simulink model "UAV_SIMULATOR_CA_2021a"  (R2024a)
settings: Solver=FixedStepAuto  StartTime=0.0  StopTime=tf_echelons  FixedStep=0.002  RelTol=1e-4
values from neighbouring files (symbols this model uses):
  Beta_OPT = [Beta, Z_max: 0.1*pi/180: betaf]    [UAV_SIMULATOR_MAIN_0.m]
  betaf = 20*pi/180 +betai    (= 0.660268528005)    [UAV_SIMULATOR_MAIN_0.m]
  betai = 17.8306*pi/180    (= 0.311202677606)    [UAV_SIMULATOR_MAIN_0.m]
  Bp_offset = 0.06    [UAV_SIMULATOR_MAIN_0.m]
  CDy = data(1)    [Aero_initial.m]    (also in FunLagragian.m; UAV_SIMULATOR_MAIN_0.m = 1; costFunction.m; nonLinearConstraints.m)
  CLOSED_LOOP_ESCs = 1    [UAV_SIMULATOR_MAIN_0.m]
  cQ = 2.1113*1e-08    (= 2.1113e-08)    [UAV_SIMULATOR_MAIN_0.m]
  cQ_Magnus = 0.5*S/2*RM^3*Cf    (= 4.804078125e-10)    [UAV_SIMULATOR_MAIN_0.m]
  cT = 2.4815e-6    (= 2.4815e-06)    [UAV_SIMULATOR_MAIN_0.m]
  cT_1_6 = 2.1030e-06    (= 2.103e-06)    [UAV_SIMULATOR_MAIN_0.m]
  D_PQR_PX4 = diag([D_ROLL D_PITCH D_YAW])    [UAV_SIMULATOR_MAIN_0.m]
  ethaf = 25*pi/180    (= 0.436332312999)    [UAV_SIMULATOR_MAIN_0.m]
  ethai = 0 *pi/180    (= 0)    [UAV_SIMULATOR_MAIN_0.m]
  F_fric = 0.5    [UAV_SIMULATOR_MAIN_0.m]
  Fa_L_int = Rmat*(FaG_int+FaG_int_d)    [UAV_SIMULATOR_MAIN_0.m]
  g = data(7)    [FunLagragian.m]    (also in UAV_SIMULATOR_MAIN_0.m = 9.81; costFunction.m; nonLinearConstraints.m; runOptimizationHelper.m = comp(7))
  I_PQR_PX4 = diag([I_ROLL I_PITCH I_YAW])    [UAV_SIMULATOR_MAIN_0.m]
  initial_attitude_condition = 1*[0 0 pi]    [UAV_SIMULATOR_MAIN_0.m]
  initial_pos_conditions = [ri*cos(betai) 0 ri*sin(betai) + Bp_offset]    [UAV_SIMULATOR_MAIN_0.m]
  Jr = 1.2991*1e-05    (= 1.2991e-05)    [UAV_SIMULATOR_MAIN_0.m]
  Jr_Magnus = JM1(2,2)    [UAV_SIMULATOR_MAIN_0.m]
  K_DI_int = [diag([k_r(1), k_etha(1), k_beta(1)]), diag([k_r(2), k_etha(2), k_beta(2)]), diag([k_r(3), k_etha(3), k_beta(3)])]    [UAV_SIMULATOR_MAIN_0.m]
  K_PQR_PX4 = 1*diag([0.8 1.35 1])    [UAV_SIMULATOR_MAIN_0.m]
  km = 1/Kv_motor_rad    (= 0.00545674090601)    [UAV_SIMULATOR_MAIN_0.m]
  L = lqr(A,B,Q_beta,R_beta)    [UAV_SIMULATOR_MAIN_0.m]
  L_mot = 1.0000e-04    (= 0.0001)    [UAV_SIMULATOR_MAIN_0.m]
  LM = 0.28*2    (= 0.56)    [UAV_SIMULATOR_MAIN_0.m]
  m = data(6)    [FunLagragian.m]    (also in UAV_SIMULATOR_MAIN_0.m = 1.746; costFunction.m; nonLinearConstraints.m; runOptimizationHelper.m = comp(6))
  m_M1 = 0.049    [UAV_SIMULATOR_MAIN_0.m]
  m_M2 = 0.049    [UAV_SIMULATOR_MAIN_0.m]
  m_w = 0.0481    [UAV_SIMULATOR_MAIN_0.m]    (also in nonLinearConstraints.m = data(9); runOptimizationHelper.m = comp(9))
  max_angle = max_angle_deg*pi/180    (= 0.610865238198)    [UAV_SIMULATOR_MAIN_0.m]
  nb_battery_cells = 4    [UAV_SIMULATOR_MAIN_0.m]
  P_ATTITUDE_PX4 = diag([10 10 2.8])    [UAV_SIMULATOR_MAIN_0.m]
  P_PQR_PX4 = diag([P_ROLL P_PITCH P_YAW])    [UAV_SIMULATOR_MAIN_0.m]
  PX4_attitude_loop_frequency = 250    [UAV_SIMULATOR_MAIN_0.m]
  PX4_rate_loop_frequency = 500    [UAV_SIMULATOR_MAIN_0.m]
  R = data(4)    [Aero_initial.m]    (also in UAV_SIMULATOR_MAIN_0.m = 0.07)
  R_bat = 0.024    [UAV_SIMULATOR_MAIN_0.m]
  rf = 1.5    [UAV_SIMULATOR_MAIN_0.m]
  rho_air = data(8)    [FunLagragian.m]    (also in UAV_SIMULATOR_MAIN_0.m = 1.293; costFunction.m; nonLinearConstraints.m; runOptimizationHelper.m = comp(8))
  ri = 0.490142    [UAV_SIMULATOR_MAIN_0.m]
  RM = data(4)    [FunLagragian.m]    (also in UAV_SIMULATOR_MAIN_0.m = 0.0275; costFunction.m; nonLinearConstraints.m; runOptimizationHelper.m = comp(4))
  S = data(3)    [Aero_initial.m]    (also in FunLagragian.m; UAV_SIMULATOR_MAIN_0.m = 0.0308; costFunction.m; nonLinearConstraints.m)
  s_M1D = [0, LM/4, 0]'    [UAV_SIMULATOR_MAIN_0.m]
  s_M2D = [0, -LM/4, 0]'    [UAV_SIMULATOR_MAIN_0.m]
  Slat = data(2)    [Aero_initial.m]    (also in FunLagragian.m; UAV_SIMULATOR_MAIN_0.m = 0.00237582944428; costFunction.m; nonLinearConstraints.m)
  state_int = [0 0 0 initial_attitude_condition 0 0 0 initial_attitude_quaternion_condition]    [UAV_SIMULATOR_MAIN_0.m]
  T0 = 1.5    [UAV_SIMULATOR_MAIN_0.m]
  t0 = 0    [UAV_SIMULATOR_MAIN_0.m]
  t1 = t0 + 15    (= 15)    [UAV_SIMULATOR_MAIN_0.m]
  t1T = t1/10    (= 1.5)    [UAV_SIMULATOR_MAIN_0.m]
  t2 = t1 + 15    (= 30)    [UAV_SIMULATOR_MAIN_0.m]    (also in plot_test.m = Simulation_Data.time)
  t2T = t2 + 9*t1/10    (= 43.5)    [UAV_SIMULATOR_MAIN_0.m]
  t3 = t2 + 15    (= 45)    [UAV_SIMULATOR_MAIN_0.m]
  tau_ur_model = 0.001    [UAV_SIMULATOR_MAIN_0.m]
  Tf = 1.5    [UAV_SIMULATOR_MAIN_0.m]
  Ti = 0    [UAV_SIMULATOR_MAIN_0.m]
  Ts = 0.02    [UAV_SIMULATOR_MAIN_0.m]
  U_sat = 3.7*nb_battery_cells    (= 14.8)    [UAV_SIMULATOR_MAIN_0.m]
  ViconTracker_noise_mean = 0.00001    (= 1e-05)    [UAV_SIMULATOR_MAIN_0.m]
  ViconTracker_noise_variance = 0.000001    (= 1e-06)    [UAV_SIMULATOR_MAIN_0.m]
  vitesse_vent = [0, 0, 0]'    [UAV_SIMULATOR_MAIN_0.m]
  vmag = 0    [UAV_SIMULATOR_MAIN_0.m]
  vx_wind = [vwind(1,1:t_winddirc_change/dt-1) vx_inter vwind(1,(t_winddirc_change+1)/dt +1:final_time/dt+1)*cos(10*pi/180)]    [UAV_SIMULATOR_MAIN_0.m]
  vy_wind = [zeros(1,t_winddirc_change/dt-1) vy_inter vwind(1,(t_winddirc_change+1)/dt +1:final_time/dt+1)*sin(10*pi/180)]    [UAV_SIMULATOR_MAIN_0.m]
  wind_turb = 1    [UAV_SIMULATOR_MAIN_0.m]
  wn_beta = 2    [UAV_SIMULATOR_MAIN_0.m]
  wn_etha = 2    [UAV_SIMULATOR_MAIN_0.m]
  wn_r = 2    [UAV_SIMULATOR_MAIN_0.m]
  X0 = 4    [UAV_SIMULATOR_MAIN_0.m]    (also in runOptimizationHelper.m = data(19))
  X1 = min(X1,8)    [Aero_initial.m]    (also in UAV_SIMULATOR_MAIN_0.m = [X1, X1(end)])
undefined symbols (not defined in the file or in its folder): DiscIntNeverNeededParam, PWM_data_map
libraries: simulink x23, slpidlib x5, eeGeneralControl x3, simulink_extras x1
(part 1 of 3)
settings Model: Creator=admin  LastModifiedBy=Abdelateef
settings DataIOCC: ReturnWorkspaceOutputs=off
settings DebuggingCC: UnconnectedInputMsg=warning  UnconnectedOutputMsg=warning  UnconnectedLineMsg=warning  ArithmeticOperatorsInVariantConditions=warning
settings ModelReferenceCC: EnableRefExpFcnMdlSchedulingChecks=on
settings SFSimCC: SimCustomHeaderCode=calculateOptimizedMagnusAndResidualForces.h  SimParseCustomCode=off  CustomCodeUndefinedFunction=UseInterfaceOnly
settings RTWCC: GPUComputeCapability=3.5  DLArmComputeVersion=19.05

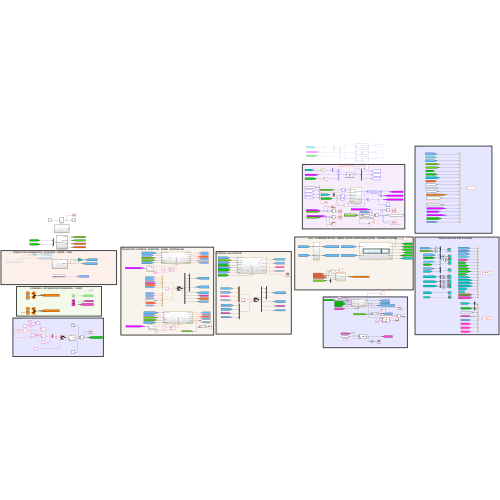
[thumbnail: Simulink's stored preview of the top-level diagram]
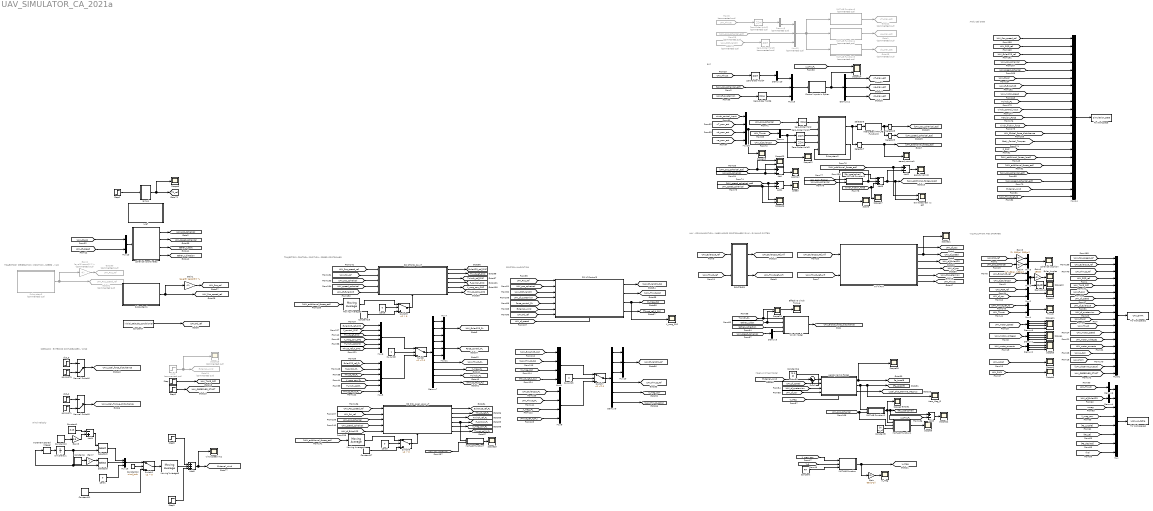
== system UAV_SIMULATOR_CA_2021a ==
  note: Analyzed Data
  note: Magnus Wings Model
  note: TRAJECTORY GENERATION : POSITION - SPEED - YAW
  note: SCENARIO : EXTERIOR DISTURBANCES - WIND
  note: TRAJECTORY CONTROL: POSITION - SPEED CONTROLLER
  note: UAV : COMMUNICATION - INNER LOOPS CONTROLLERS (PX4) - DYNAMIC SYSTEM
  note: VIZUALIZATION AND STORAGE
  note: EKF
  note: CONTROL ALLOCATION
  note: Wind Velocity
  2D LF Control3 : Subsystem
      settings: PortSchema="{\"entries\":[{\"content\":{\"sides\":[{\"content\":{\"connectorIds\":[\"In1\",\"In2\",\"In3\",\"In4\",\"In5\",\"In6\",\"In7\"]},\"type\":\"ConnectorPlacement.EquallySpacedRectSide\",\"uuid\":\"a86b3051-01d7-4a85-8d20-3f69d77c03a1\"},{\"content\":{\"connectorIds\":[\"Out1\",\"Out2\",\"Out3\",\"Out4\"],\"side\":\"RIGHT\"},\"type\":\"ConnectorPlacement.EquallySpacedRectSide\",\"uuid\":\"bc9590fb-a9f5-4f22-833c-6f7b6fce8796\"},{\"content\":{\"connectorIds\":[],\"side\":\"TOP\"},\"type\":\"ConnectorPlacement.EquallySpacedRectSide\",\"uuid\":\"ed461341-60ff-412b-af3b-1b94a2f94912\"},{\"content\":{\"connectorIds\":[\"In8\"],\"side\":\"BOTTOM\"},\"type\":\"ConnectorPlacement.EquallySpacedRectSide\",\"uuid\":\"06185854-d4ab-4a15-925c-b5ae7d14fbfc\"}]},\"type\":\"ConnectorPlacement.EquallySpacedConnector\",\"uuid\":\"5ffbe6af-ef45-41d3-b7b2-7d73faf302ea\"}],\"packageUris\":[\"http://schema.mathworks.com/mf0/Connector/R2020b\"],\"version\":\"1.0\"}"
  3D PID- open Loop uT : Subsystem
      settings: PortSchema="{\"entries\":[{\"content\":{\"sides\":[{\"content\":{\"connectorIds\":[\"In1\",\"In2\",\"In3\",\"In4\",\"In5\"]},\"type\":\"ConnectorPlacement.EquallySpacedRectSide\",\"uuid\":\"61a30ab6-05c4-4e42-9f51-0dbdd622c055\"},{\"content\":{\"connectorIds\":[\"Out1\",\"Out2\",\"Out3\",\"Out4\",\"Out5\",\"Out6\"],\"side\":\"RIGHT\"},\"type\":\"ConnectorPlacement.EquallySpacedRectSide\",\"uuid\":\"1c2ba6ee-e8e1-4086-9bbe-d900aead1114\"},{\"content\":{\"connectorIds\":[],\"side\":\"TOP\"},\"type\":\"ConnectorPlacement.EquallySpacedRectSide\",\"uuid\":\"9ceaf1b7-f62f-4f6d-a488-9bf5cd150116\"},{\"content\":{\"connectorIds\":[\"In6\"],\"side\":\"BOTTOM\"},\"type\":\"ConnectorPlacement.EquallySpacedRectSide\",\"uuid\":\"50e45314-3425-4ab8-8018-46313f9291af\"}]},\"type\":\"ConnectorPlacement.EquallySpacedConnector\",\"uuid\":\"bdde6506-7878-4542-8fe8-5fcc1ce9dea7\"}],\"packageUris\":[\"http://schema.mathworks.com/mf0/Connector/R2020b\"],\"version\":\"1.0\"}"
  3D STSMC- CA uT : Subsystem
      settings: PortSchema="{\"entries\":[{\"content\":{\"sides\":[{\"content\":{\"connectorIds\":[\"In1\",\"In2\",\"In3\",\"In4\",\"In5\"]},\"type\":\"ConnectorPlacement.EquallySpacedRectSide\",\"uuid\":\"61a30ab6-05c4-4e42-9f51-0dbdd622c055\"},{\"content\":{\"connectorIds\":[\"Out1\",\"Out2\",\"Out3\",\"Out4\",\"Out5\",\"Out6\"],\"side\":\"RIGHT\"},\"type\":\"ConnectorPlacement.EquallySpacedRectSide\",\"uuid\":\"1c2ba6ee-e8e1-4086-9bbe-d900aead1114\"},{\"content\":{\"connectorIds\":[],\"side\":\"TOP\"},\"type\":\"ConnectorPlacement.EquallySpacedRectSide\",\"uuid\":\"9ceaf1b7-f62f-4f6d-a488-9bf5cd150116\"},{\"content\":{\"connectorIds\":[\"In6\"],\"side\":\"BOTTOM\"},\"type\":\"ConnectorPlacement.EquallySpacedRectSide\",\"uuid\":\"50e45314-3425-4ab8-8018-46313f9291af\"}]},\"type\":\"ConnectorPlacement.EquallySpacedConnector\",\"uuid\":\"bdde6506-7878-4542-8fe8-5fcc1ce9dea7\"}],\"packageUris\":[\"http://schema.mathworks.com/mf0/Connector/R2020b\"],\"version\":\"1.0\"}"
  Add{,1..3} (4 alike) : Sum  Inputs=+-
  Add4 : Sum  Inputs=-+
  Add5 : Sum  Inputs=++-
  Add6 : Sum  Inputs=+++
  Aero_Mag_G : Scope
  Aerodynamic Forces : Subsystem
      settings: PortSchema="{\"entries\":[{\"content\":{\"sides\":[{\"content\":{\"connectorIds\":[\"In1\",\"In2\",\"In3\",\"In4\"]},\"type\":\"ConnectorPlacement.EquallySpacedRectSide\",\"uuid\":\"3316b48e-b4d5-45c4-9d90-a617ed73544d\"},{\"content\":{\"connectorIds\":[\"Out1\",\"Out2\",\"Out3\"],\"side\":\"RIGHT\"},\"type\":\"ConnectorPlacement.EquallySpacedRectSide\",\"uuid\":\"a0895ec7-47a4-40cb-908f-8eab4289e36a\"},{\"content\":{\"connectorIds\":[],\"side\":\"TOP\"},\"type\":\"ConnectorPlacement.EquallySpacedRectSide\",\"uuid\":\"7ad0bb64-841b-42b9-aa6a-2e12b7a3b2cf\"},{\"content\":{\"connectorIds\":[\"In5\"],\"side\":\"BOTTOM\"},\"type\":\"ConnectorPlacement.EquallySpacedRectSide\",\"uuid\":\"cbeb3cbb-bd59-4a2c-a4ec-b6bf92c1c233\"}]},\"type\":\"ConnectorPlacement.EquallySpacedConnector\",\"uuid\":\"e2406028-c72c-44a7-a706-79825605090e\"}],\"packageUris\":[\"http://schema.mathworks.com/mf0/Connector/R2020b\"],\"version\":\"1.0\"}"
  CA switch : Constant  Value=0
  Constant : Constant  Value=RM
  Constant1 : Constant  Value=8.25
  Constant10 : Constant  Value=vx_wind
  Constant11 : Constant  Value=[vmag 0 0]
  Constant12 : Constant  Value=wind_turb
  Constant16 : Constant  Value=[0 0 0]
  Constant17 : Constant  Value=[0;0;0]
  Constant18 : Constant  Value=[0;0;0]
  Constant4 : Constant  Value=vy_wind
  Constant7 : Constant  Value=initial_attitude_condition(3)
  Constant9 : Constant  Value=[m m_w]
  Control Inputs in Spher : MATLAB Function  TreatAsAtomicUnit=on
  Demux{,3..4,6,10..11} (6 alike) : Demux  Outputs=3
  Demux1 : Demux
  Demux2 : Demux
  Demux5 : Demux
  Demux7 : Demux  Outputs=10
  Demux8 : Demux  Commented=on  Outputs=3
  Demux9 : Demux  Outputs=6
  Derivative : Derivative
  Effective winch Torque : Scope
  Euler_Angles : Scope
  From28 : From  Commented=on  GotoTag=UAV_pos_spherical_est
  From5 : From  Commented=on  GotoTag=UAV_Thrust  TagVisibility=global
  From73 : From  Commented=on  GotoTag=UAV_sf_Euler123  TagVisibility=global
  Gain : Gain  Gain=60/(2*pi)
  Gain1 : Gain  Gain=[eye(3) zeros(3) ]  Multiplication=Matrix(K*u) (u vector)
  Gain2 : Gain  Commented=on  Gain=[eye(3) zeros(3) ]  Multiplication=Matrix(K*u) (u vector)
  Gain3 : Gain  Gain=[1, 180/pi, 180/pi]
  Gain4 : Gain  Gain=[1, 180/pi, 180/pi]
  Gain5 : Gain  Gain=1.5
  Gain6 : Gain  Gain=180/pi
  Gain7 : Gain
  Goto1 : Goto  Commented=on  GotoTag=ue_prev_est  TagVisibility=global
  Goto15 : Goto  Commented=on  GotoTag=ub_prev_est  TagVisibility=global
  Goto22 : Goto  Commented=on  GotoTag=uT_prev_est  TagVisibility=global
  Goto24 : Goto  Commented=on  GotoTag=External_wind  TagVisibility=global
  Goto90 : Goto  Commented=on  GotoTag=UAV_Pos_ref  TagVisibility=global
  Goto91 : Goto  Commented=on  GotoTag=UAV_Pos_speed_ref  TagVisibility=global
  Increment Stored Integer : simulink/Additional Math & Discrete/Additional Math: Increment - Decrement/Increment Stored Integer
  Interpreted MATLAB Function3 : MATLABFcn  MATLABFcn=[u(1); u(3); u(5); u(2); u(4); u(6)]  OutputDimensions=6
  MATLAB Function : MATLAB Function  TreatAsAtomicUnit=on
  MATLAB Function1 : MATLAB Function  TreatAsAtomicUnit=on
  MATLAB Function2 : MATLAB Function  TreatAsAtomicUnit=on
  MATLAB Function3 : MATLAB Function  TreatAsAtomicUnit=on
  MATLAB Function4 : MATLAB Function  Commented=on  TreatAsAtomicUnit=on
  MATLAB Function5 : MATLAB Function  Commented=on  TreatAsAtomicUnit=on
  MATLAB Function6 : MATLAB Function  Commented=on  TreatAsAtomicUnit=on
  MATLAB Function7 : MATLAB Function  TreatAsAtomicUnit=on
  Manual Switch5 : ManualSwitch  CurrentSetting=0
  Manual Switch6 : ManualSwitch  CurrentSetting=0
  Moving Average1 : eeGeneralControl/Moving Average  VariantControl=Variant1  LabelModeActiveChoice=Discrete  f=50  x0=0  BufferSize=8192  Ts=-1
  Moving Average2 : eeGeneralControl/Moving Average  VariantControl=Variant1  LabelModeActiveChoice=Discrete  f=50  x0=0  BufferSize=8192  Ts=-1
  Moving Average3 : eeGeneralControl/Moving Average  VariantControl=Variant1  LabelModeActiveChoice=Discrete  f=50  x0=0  BufferSize=8192  Ts=-1
  Mux : Mux  Inputs=8
  Mux{1..4,13} (5 alike) : Mux  Inputs=2
  Mux{7,10..11,15..16} (5 alike) : Mux  Inputs=3
  Mux12 : Mux  Commented=on  Inputs=3
  Mux14 : Mux  Inputs=21
  Mux26 : Mux
  Mux5 : Mux  Inputs=6
  Mux51 : Mux  Inputs=18
  Mux6 : Mux  Inputs=6
  Mux8 : Mux
  Mux9 : Mux
  NO DIST1 : Step  Time=3  After=[0 0 0]
  NO DIST3 : Step  Time=3  After=[0 0 0]
  PL switch : Constant
  ROUTEUR1 : Subsystem
  Scope{,1..3,6,8..10,12..13,17..18,20..22,25} (16 alike) : Scope
  Scope11 : Scope  NumInputPorts=4
  Scope14 : Scope  NumInputPorts=2
  Scope15 : Scope  Commented=on
  Scope23 : Scope  NumInputPorts=2
  Scope26 : Scope  NumInputPorts=2
  Scope4 : Scope  NumInputPorts=4
  Scope5 : Scope  NumInputPorts=4
  Selector2 : Selector  InputPortWidth=wind_clm  IndexOptions=Starting index (port)  Indices=[1 3]  OutputSizes=1
  Selector3 : Selector  InputPortWidth=wind_clm  IndexOptions=Starting index (port)  Indices=[1 3]  OutputSizes=1
  Selector6 : Selector  InputPortWidth=9  IndexOptions=Index vector (dialog)  Indices=[1:6]  OutputSizes=1
  Selector7 : Selector  InputPortWidth=9  IndexOptions=Index vector (dialog)  Indices=[7:9]  OutputSizes=1
  Selector8 : Selector  InputPortWidth=6  IndexOptions=Index vector (dialog)  Indices=[1:3]  OutputSizes=1
  Selector9 : Selector  InputPortWidth=6  IndexOptions=Index vector (dialog)  Indices=[4:6]  OutputSizes=1
  Step : Step  Time=0  SampleTime=0
  Step1 : Step  Time=0  SampleTime=0
  Step2 : Step  Time=0  SampleTime=0
  Step3 : Step  Time=20  Before=[0, 0, 0]  After=[3, 0, 0]  SampleTime=0
  Step5 : Step  Time=0.017  Before=[3.3, 0, 0]  After=0  SampleTime=0
  Subsystem1 : Subsystem
  Subsystem2 : Subsystem
  Subsystem3 : Subsystem  Commented=on
  Sum1 : Sum  Inputs=|+-
  Switch : Switch  Criteria=u2 ~= 0  Threshold=0.5  SaturateOnIntegerOverflow=off  InputSameDT=off
  Switch2 : Switch  Criteria=u2 > Threshold  SaturateOnIntegerOverflow=off  InputSameDT=off
  Switch7 : Switch  Criteria=u2 ~= 0  Threshold=0.5  SaturateOnIntegerOverflow=off  InputSameDT=off
  Switch8 : Switch  Criteria=u2 > Threshold  SaturateOnIntegerOverflow=off  InputSameDT=off
  Switch9 : Switch  Criteria=u2 > Threshold  SaturateOnIntegerOverflow=off  InputSameDT=off
  Thrust : Scope
  To Workspace : ToWorkspace  VariableName=Simulation_Data  SaveFormat=Structure With Time  SampleTime=-1
  To Workspace1 : ToWorkspace  VariableName=UAV_DATA  SaveFormat=Timeseries  SampleTime=-1
  To Workspace2 : ToWorkspace  VariableName=Look_up_table  SaveFormat=Structure With Time  SampleTime=-1
  Unit Delay1 : UnitDelay  InitialCondition=1  SampleTime=-1  HasFrameUpgradeWarning=on
  Winch Model : Subsystem
  "X4 + PX4 " : Subsystem
  X_mag_CA2 : Scope
  Zero-Order Hold{,1,3..4,6} (5 alike) : ZeroOrderHold  SampleTime=Ts
  Zero-Order Hold2 : ZeroOrderHold  Commented=on  SampleTime=Ts
  Zero-Order Hold5 : ZeroOrderHold  Commented=on  SampleTime=Ts
  Zero1 : Constant  Value=0  OutDataTypeStr=Inherit: Inherit via back propagation
  Zero5 : Constant  Value=0  OutDataTypeStr=Inherit: Inherit via back propagation
  Zero8 : Constant  Value=0  OutDataTypeStr=Inherit: Inherit via back propagation
  aerodynamics : Scope
  aerodynamics1 : Scope
  dist_2 : Step  Time=10  After=[0 0 0]
  dist_3 : Step  Time=10  After=[0 1 0]
  ext forces real vs est : Scope  NumInputPorts=2
  position : Scope
  r_ref : Subsystem
  ramp4 : Subsystem  mask{tf1=2, tf2=24+34-2*2, tf3=2, g1=T0/2, g2=T0/2}
      mask prompts: tf1 "temps fin rampe montante"; tf2 "temps fin constante"; tf3 "temps fin rampe descendente"; g1 "gain rampe 1"; g2 "gain rampe 2"
  speed : Scope
  spherical coordinates : Subsystem
  spherical position : Scope
  w_Mag : Scope
  wind : Step  Commented=on  Time=0  Before=[ 0 0 0]  After=vitesse_vent
  wind speed m/s : Scope
  tag scope: Euler123_ref_FL=global, Euler123_ref_SMC=global, External_wind=global, F_control_FL=global, F_control_SMC=global, Fa_LocalB=global, Force_control_PL=global, Local_Dist_Gamma_Magnus=global, T0_ref=global, Thrust_ref_FL=global, Thrust_ref_N_FL=global, Thrust_ref_N_SMC=global, Thrust_ref_SMC=global, Twinch_PL=global, Twinch_ref_FL=global, Twinch_ref_SMC=global, UAV_Euler123_PL=global, UAV_Euler123_ref=global, UAV_Euler123_ref_wifi=global, UAV_Global_force_disturbance=global, UAV_Local_Torque_Disturbance=global, UAV_Local_force_disturbance=global, UAV_OBSERVER_START=global, UAV_Pos_ref=global, UAV_Pos_speed_ref=global, UAV_Psi_ref=global, UAV_TAKE_OFF=global, UAV_Thrust=global, UAV_Thrust_PL=global, UAV_Thrust_ref=global, UAV_Thrust_ref_wifi=global, UAV_pos_spherical=global, UAV_sf_Euler123=global, UAV_sf_pos=global, UAV_sf_pqr=global, UAV_sf_quaternion=global, UAV_sf_speed=global, UAV_speed_spherical=global, X_mag_PL=global, X_mag_corr=global, X_mag_corr_FL=global, X_mag_corr_SMC=global, tether_r_ddot=global, tether_r_direction=global, uT_prev_est=global, ub_prev_est=global, ue_prev_est=global, w_Mag=global
  wires:
  Demux5/1 -> Scope11/1  "Motor1"
  Demux5/2 -> Scope11/2  "Motor2"
  Demux5/3 -> Scope11/3  "Motor3"
  Demux5/4 -> Scope11/4  "Motor4"
  Gain3/1 -> Mux3/1
  Manual Switch5/1 -> [UAV_Local_Torque_Disturbance]  "dist_Gamma_pqr_Thrust"
  Gain4/1 -> Mux3/2
  [UAV_motor_speed] -> Demux5/1
  NO DIST3/1 -> Manual Switch6/2
  Manual Switch6/1 -> [UAV_Local_force_disturbance]  "dist_Gamma_pqr_Thrust"
  dist_3/1 -> Manual Switch6/1
  [UAV_Thrust_ref] -> ROUTEUR1/2(In2)
  [UAV_Euler123_ref] -> ROUTEUR1/1(In1)
  [UAV_Euler123_ref_wifi] -> "X4 + PX4 "/1(In1)
  Mux51/1 -> To Workspace1/1
  [UAV_Thrust_ref_wifi] -> "X4 + PX4 "/2(real thrust)
  [UAV_sf_Euler123] -> Mux1/2
  [UAV_Euler123_ref] -> Mux1/1
  Mux1/1 -> Derivative/1, Gain6/1
  Mux2/1 -> Scope2/1
  Demux1/4 -> Scope4/4  "Motor4"
  Demux1/3 -> Scope4/3  "Motor3"
  Demux1/2 -> Scope4/2  "Motor2"
  Demux1/1 -> Scope4/1  "Motor1"
  Demux2/1 -> Scope5/1  "Motor1"
  Demux2/2 -> Scope5/2  "Motor2"
  Demux2/3 -> Scope5/3  "Motor3"
  Demux2/4 -> Scope5/4  "Motor4"
  [UAV_motor_currents] -> Demux2/1
  [UAV_motor_voltages] -> Demux1/1
  [UAV_U_bat] -> Scope3/1
  [UAV_PWM] -> Scope6/1
  dist_2/1 -> Manual Switch5/1
  NO DIST1/1 -> Manual Switch5/2
  Mux4/1 -> Thrust/1
  [UAV_Pos_speed_ref] -> Mux51/1
  [UAV_Euler123_ref] -> Mux51/2
  [UAV_Thrust_ref] -> Mux51/3
  [UAV_PQR_ref] -> Mux51/4
  [UAV_TAKE_OFF] -> Mux51/5
  [UAV_sf_pos] -> Mux51/6
  [UAV_sf_speed] -> Mux51/7
  [UAV_sf_Euler123] -> Mux51/8
  [UAV_sf_quaternion] -> Mux51/9
  [UAV_sf_pqr] -> Mux51/10
  [UAV_Thrust] -> Mux51/11
  [UAV_motor_speed] -> Mux51/12
  [UAV_motor_voltages] -> Mux51/13
  [UAV_motor_currents] -> Mux51/14
  [UAV_U_bat] -> Mux51/15
  [UAV_PWM] -> Mux51/16
  Step/1 -> [UAV_TAKE_OFF]
  Step2/1 -> [UAV_OBSERVER_START]
  [UAV_observer_output] -> Mux51/17
  [UAV_OBSERVER_START] -> Mux51/18
  [UAV_Thrust] -> Mux4/2
  [UAV_sf_speed] -> Aerodynamic Forces/2(u)  "V_drone"
  Aerodynamic Forces/3(Gamma) -> [Local_Dist_Gamma_Magnus]
  Sum1/1 -> Aerodynamic Forces/1(In1)  "external wind m/s"
  [UAV_sf_quaternion] -> Aerodynamic Forces/3(quad)  "quaternion"
  Aerodynamic Forces/1(Output) -> Scope18/1, [Fa_LocalB]
  [UAV_sf_pqr] -> Aerodynamic Forces/4(In4)  "pqr"
  [w_Mag] -> Aerodynamic Forces/5(In5)  "spin_ratio"
  [UAV_PQR_ref] -> Mux2/1
  [UAV_sf_pqr] -> Mux2/2
  [X_mag_corr] -> MATLAB Function/1(X)  "spin_ratio"
  [V_a] -> MATLAB Function/2(Va)
  Constant/1 -> MATLAB Function/3(RM)
  Gain/1 -> w_Mag/1
  [UAV_sf_Euler123] -> Demux4/1
  Mux/1 -> To Workspace2/1
  Demux4/2 -> Mux/2
  [wmag] -> Mux/3
  [X_mag_corr] -> Mux/4  "spin_ratio"
  [UAV_Thrust] -> Demux6/1
  Gain6/1 -> Euler_Angles/1
  Demux6/3 -> Mux/1
  Demux7/3 -> Mux7/3
  [Euler123_ref_FL] -> Mux5/1
  Demux7/1 -> Mux7/1
  [Euler123_ref_SMC] -> Mux6/1
  Demux7/2 -> Mux7/2
  PL switch/1 -> Switch/2
  Mux6/1 -> Switch/1
  Mux5/1 -> Switch/3
  Mux7/1 -> [UAV_Euler123_PL]
  Derivative/1 -> Scope10/1
  [Fa_LocalG] -> Mux/5
  [Fa_LG] -> Mux/6
  [FG_desired] -> Mux/7
  [UAV_Thrust_ref_N] -> Mux4/1
  MATLAB Function/1(w_ref) -> [w_Mag], Gain/1
  [fval] -> Mux/8
  [tether_r_ddot] -> Scope20/1, Winch Model/2(r_ddot)
  [tether_r_direction] -> Winch Model/3(r_dir)
  Demux3/1 -> Winch Model/4(r_dot)
  [UAV_speed_spherical] -> Demux3/1
  Winch Model/1(T_tether) -> [UAV_Global_force_disturbance]
  Mux13/1 -> spherical coordinates/1("cartesian position ")
  [UAV_sf_pos] -> Mux13/1
  spherical coordinates/2(speed_spher) -> [UAV_speed_spherical]
  spherical coordinates/3(r_ddot) -> [tether_r_ddot]
  spherical coordinates/4(r_dir) -> [tether_r_direction]
  [UAV_sf_speed] -> Mux13/2
  Subsystem1/1(spherical_ref) -> Gain1/1, [UAV_Pos_speed_ref]  "[pos] ref"
  Gain1/1 -> [UAV_Pos_ref]
  Constant7/1 -> [UAV_Psi_ref]
  Subsystem2/1(x_est) -> Selector7/1, Selector6/1
  Add2/1 -> aerodynamics/1
  Selector6/1 -> Interpreted MATLAB Function3/1
  Selector9/1 -> [UAV_speed_spherical_est]
  [UAV_pos_spherical_est] -> Scope23/1, Add/1
  MATLAB Function4/1(ue_prev) -> Goto1/1
  [uT_prev_est] -> Mux26/2
  Mux12/1 -> MATLAB Function5/1(input), MATLAB Function4/1(input), MATLAB Function6/1(input)
  Demux8/3 -> Mux12/1
  Add1/1 -> speed/1
  Subsystem2/2(Cov) -> Subsystem2/5(cov)
  Add/1 -> position/1
  [ue_prev_est] -> Mux26/4
  [Fa_Localspher] -> Add5/1
  [ub_prev_est] -> Mux26/3
  [UAV_speed_spherical] -> Scope26/2, Add1/2
  Interpreted MATLAB Function3/1 -> Selector8/1, Selector9/1
  Selector8/1 -> [UAV_pos_spherical_est]
  Add5/1 -> ext forces real vs est/2, [UAV_additional_forces_local], Add2/2
  [UAV_pos_spherical] -> Scope23/2, Add/2
  Mux26/1 -> Scope13/1, Subsystem2/2(control)  "control"
  [UAV_speed_spherical_est] -> Scope26/1, Add1/1
  [winch_friction_force] -> Scope17/1, Add5/3
  MATLAB Function6/1(uT0_prev) -> Goto22/1
  [winch_control_input] -> Mux26/1
  MATLAB Function5/1(ub_prev) -> Goto15/1
  [UAV_Thrust] -> Demux/1
  From5/1 -> Zero-Order Hold2/1
  From73/1 -> Zero-Order Hold5/1
  [UAV_pos_spherical] -> Zero-Order Hold/1
  [UAV_sf_Euler123] -> Zero-Order Hold3/1
  [UAV_additional_forces_est] -> ext forces real vs est/1, Add2/1
  wind/1 -> Scope15/1, Goto24/1
  Zero-Order Hold/1 -> Subsystem2/1(y)
  Zero-Order Hold1/1 -> Subsystem2/3(Thrust_ref)
  Zero-Order Hold3/1 -> Subsystem2/4(euler_ref)
  Zero-Order Hold2/1 -> Demux8/1
  From28/1 -> Mux12/2
  Zero-Order Hold5/1 -> Mux12/3
  spherical coordinates/1(pos_spher) -> [UAV_pos_spherical]
  Switch/1 -> Demux7/1
  [UAV_pos_spherical] -> MATLAB Function1/2(x), MATLAB Function2/2(data)
  Aerodynamic Forces/2(Output1) -> MATLAB Function2/1(Fa_G), Aero_Mag_G/1, [Fa_LocalG]
  MATLAB Function2/1(Fa_L) -> Add3/1, [Fa_Localspher], Scope1/1, MATLAB Function1/1(FaL)
  MATLAB Function1/1(u) -> Scope9/1
  Constant9/1 -> MATLAB Function1/3(data)
  Demux9/5 -> [X_mag_corr]
  Switch7/1 -> Demux9/1
  Mux10/1 -> [UAV_Euler123_ref]
  [UAV_Thrust_PL] -> Mux8/2
  [X_mag_PL] -> Mux8/3
  Mux8/1 -> Switch7/3
  Mux9/1 -> Switch7/1
  CA switch/1 -> Switch7/2
  Demux9/4 -> [UAV_Thrust_ref]
  Demux9/2 -> Mux10/2
  Demux9/1 -> Mux10/1
  [UAV_Euler123_PL] -> Mux8/1
  Demux9/3 -> Mux10/3
  [Twinch_ref_SMC] -> Mux6/5
  [X_mag_corr_SMC] -> Mux6/4
  [Thrust_ref_SMC] -> Mux6/3
  [F_control_SMC] -> Mux6/2
  [Twinch_ref_FL] -> Mux5/5
  [X_mag_corr_FL] -> Mux5/4
  [Thrust_ref_FL] -> Mux5/3
  [F_control_FL] -> Mux5/2
  Demux7/4 -> Mux11/1
  Demux7/5 -> Mux11/2
  Demux7/6 -> Mux11/3
  Demux7/9 -> [Twinch_PL]
  Demux7/8 -> [X_mag_PL]
  Demux7/7 -> [UAV_Thrust_PL]
  Mux11/1 -> [Force_control_PL]
  [UAV_Thrust_CA] -> Mux9/2
  [UAV_Euler123_CA] -> Mux9/1
  [X_mag_CA] -> Mux9/3
  "X4 + PX4 "/1(Out5) -> [UAV_sf_pos]
  "X4 + PX4 "/2(Out6) -> Scope21/1, [UAV_sf_speed]
  "X4 + PX4 "/4(Out8) -> [UAV_sf_pqr]
  "X4 + PX4 "/5(Out1) -> [UAV_sf_quaternion]
  "X4 + PX4 "/6(Out2) -> [UAV_Thrust]
  "X4 + PX4 "/3(Out7) -> [UAV_sf_Euler123]
  [Thrust_ref_N_SMC] -> Mux6/6
  [Thrust_ref_N_FL] -> Mux5/6
  Demux7/10 -> [Thrust_ref_N_PL]
  [Thrust_ref_N_PL] -> Mux8/4
  [Thrust_ref_N_CA] -> Mux9/4
  Demux9/6 -> [UAV_Thrust_ref_N]
  Mux3/1 -> spherical position/1
  [UAV_Pos_ref] -> Gain3/1
  [UAV_pos_spherical] -> Gain4/1
  [UAV_pos_spherical] -> MATLAB Function3/2(data)
  [UAV_aero_Global] -> MATLAB Function3/1(Fa_G)
  MATLAB Function3/1(Fa_L) -> Scope/1, Add5/2
  ramp4/1(Out1) -> Scope8/1, [T0_ref]
  Add4/1 -> Selector2/1
  Mux16/1 -> Switch2/1
  Constant12/1 -> Switch2/2
  Unit Delay1/1 -> Increment Stored Integer/1, Selector3/2, Selector2/2
  Zero1/1 -> Mux16/3
  Constant4/1 -> Gain7/1
  Constant11/1 -> Switch2/3
  Increment Stored Integer/1 -> Unit Delay1/1
  Selector3/1 -> Mux16/2
  Selector7/1 -> aerodynamics1/1, [UAV_additional_forces_est]
  Demux/3 -> Scope12/1, Zero-Order Hold1/1
  [Twinch_PL] -> Effective winch Torque/1, Winch Model/1(u_r)
  [UAV_sf_speed] -> 2D LF Control3/8(In8)
  [Force_control_PL] -> 2D LF Control3/5(Euler1)
  [UAV_pos_spherical] -> 2D LF Control3/2(In1)
  [UAV_Psi_ref] -> 2D LF Control3/7(psi1)
  [UAV_sf_Euler123] -> 2D LF Control3/3(In2)
  2D LF Control3/4(Thrust_ref2) -> [Thrust_ref_N_CA]
  2D LF Control3/3(output2) -> X_mag_CA2/1, [X_mag_CA]
  [UAV_Pos_ref] -> 2D LF Control3/1(In3)
  [External_wind] -> 2D LF Control3/6(u)
  2D LF Control3/2(Thrust_ref1) -> [UAV_Thrust_CA]
  2D LF Control3/1(output1) -> [UAV_Euler123_CA]
  [UAV_sf_quaternion] -> 2D LF Control3/4(In5)
  [External_wind] -> Sum1/1  "external wind m/s"
  Constant16/1 -> Sum1/2  "external win m/s"
  3D PID- open Loop uT/2(Out2) -> [Thrust_ref_FL]
  Constant17/1 -> Switch8/3
  [UAV_speed_spherical] -> 3D PID- open Loop uT/4(Faero_s3)
  [UAV_Pos_speed_ref] -> 3D PID- open Loop uT/1(Faero_s1)
  3D PID- open Loop uT/5(Twinch_ref [N]2) -> [X_mag_corr_FL]  "X_corr"
  Zero5/1 -> Switch8/2
  [UAV_additional_forces_est] -> Moving Average1/1
  [UAV_sf_Euler123] -> 3D PID- open Loop uT/5(Euler1)
  3D PID- open Loop uT/3(Twinch_ref [N]) -> [Twinch_ref_FL]
  3D PID- open Loop uT/1(Out1) -> [Euler123_ref_FL]
  3D PID- open Loop uT/6(Out3) -> [Thrust_ref_N_FL]
  3D PID- open Loop uT/4(Twinch_ref [N]1) -> MATLAB Function7/1(Fa_L), [F_control_FL]
  Switch8/1 -> 3D PID- open Loop uT/6(Faero_s)
  [UAV_Psi_ref] -> 3D PID- open Loop uT/2(psi_ref2)
  [UAV_pos_spherical] -> 3D PID- open Loop uT/3(Faero_s2)
  [UAV_additional_forces_est] -> Moving Average2/1
  [UAV_Pos_speed_ref] -> 3D STSMC- CA uT/1(Faero_s1)
  [UAV_sf_Euler123] -> 3D STSMC- CA uT/5(Euler1)
  3D STSMC- CA uT/1(Out1) -> [Euler123_ref_SMC]
  3D STSMC- CA uT/4(Twinch_ref [N]1) -> [F_control_SMC]
  [UAV_pos_spherical] -> 3D STSMC- CA uT/3(Faero_s2)
  3D STSMC- CA uT/3(Twinch_ref [N]) -> [Twinch_ref_SMC]
  Constant18/1 -> Switch9/3
  Switch9/1 -> 3D STSMC- CA uT/6(Faero_s)
  [UAV_Psi_ref] -> 3D STSMC- CA uT/2(psi_ref2)
  [UAV_speed_spherical] -> 3D STSMC- CA uT/4(Faero_s3)
  3D STSMC- CA uT/6(Out3) -> [Thrust_ref_N_SMC]
  3D STSMC- CA uT/5(Twinch_ref [N]2) -> [X_mag_corr_SMC]  "X_corr"
  Zero8/1 -> Switch9/2
  3D STSMC- CA uT/2(Out2) -> [Thrust_ref_SMC]
  [u_UAV_FL] -> Add3/2
  Add3/1 -> Scope22/1
  ROUTEUR1/1(PQR_ref) -> [UAV_Euler123_ref_wifi]
  ROUTEUR1/2(PQR_ref1) -> [UAV_Thrust_ref_wifi]
  [UAV_pos_spherical] -> MATLAB Function7/2(data)
  MATLAB Function7/1(Fa_G) -> Scope25/1
  [UAV_Pos_speed_ref] -> Mux14/1
  [UAV_PQR_ref] -> Mux14/2
  [UAV_Euler123_ref] -> Mux14/3
  [UAV_pos_spherical] -> Mux14/4
  [UAV_speed_spherical] -> Mux14/5
  [UAV_sf_pqr] -> Mux14/6
  [UAV_sf_Euler123] -> Mux14/7
  [UAV_motor_speed] -> Mux14/8
  [Twinch_PL] -> Mux14/9
  [Tension_Force] -> Mux14/11
  [winch_friction_force] -> Mux14/12
  [UAV_Global_force_disturbance] -> Mux14/13
  [Body_Control_Torques] -> Mux14/14
  [winch_control_input] -> Mux14/10
  Mux14/1 -> To Workspace/1
  Gain2/1 -> Goto90/1
  Subsystem3/1(spherical_ref) -> Gain2/1, Goto91/1  "[pos] ref"
  Step1/1 -> ramp4/1(In1)
  Zero-Order Hold6/1 -> Mux15/3
  Zero-Order Hold4/1 -> Demux10/1
  [UAV_sf_quaternion] -> Zero-Order Hold6/1
  [UAV_Thrust] -> Zero-Order Hold4/1
  Demux10/3 -> Mux15/1
  Mux15/1 -> Control Inputs in Spher/1(data)
  Control Inputs in Spher/1(Fa_pher) -> Scope14/2, Demux11/1
  Demux11/3 -> [ub_prev_est]
  Demux11/1 -> [uT_prev_est]
  Demux11/2 -> [ue_prev_est]
  [UAV_pos_spherical_est] -> Mux15/2
  [u_UAV_FL] -> Scope14/1
  Add6/1 -> wind speed m/s/1, [External_wind]
  Constant10/1 -> Gain5/1
  [S_SMC] -> Mux14/15
  Gain5/1 -> Add4/2
  Constant1/1 -> Add4/1
  Gain7/1 -> Selector3/1
  Selector2/1 -> Mux16/1
  Step5/1 -> Add6/1
  Switch2/1 -> Moving Average3/1
  [UAV_additional_forces_local] -> Mux14/16
  [UAV_additional_forces_est] -> Mux14/17
  [UAV_pos_spherical_est] -> Mux14/18
  [UAV_speed_spherical_est] -> Mux14/19
  [External_wind] -> Mux14/20
  [UAV_Thrust_ref_N] -> Mux14/21
  Moving Average1/1 -> Switch8/1
  Moving Average2/1 -> Switch9/1
  Moving Average3/1 -> Add6/2
  Step3/1 -> Add6/3

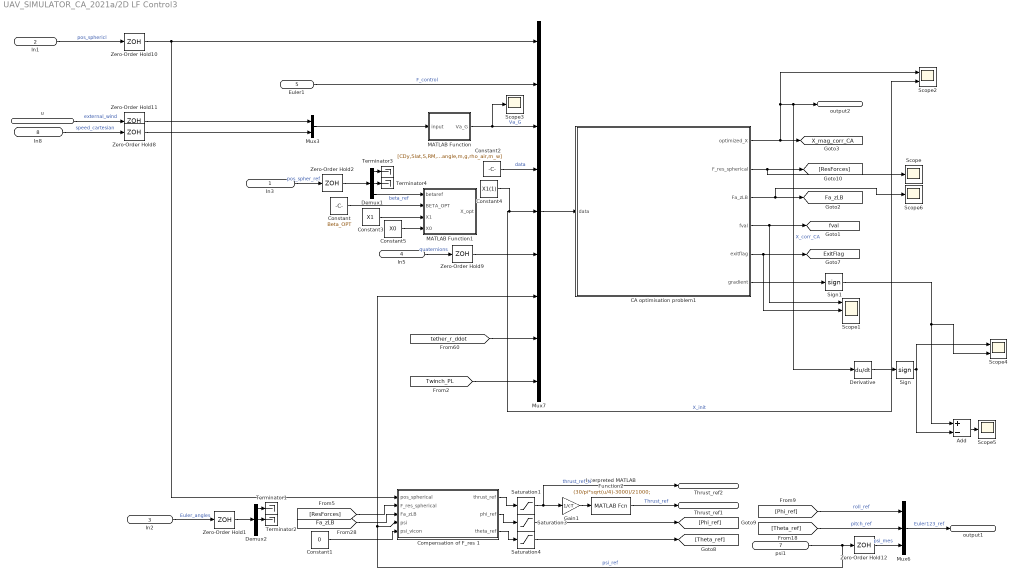
== system UAV_SIMULATOR_CA_2021a/2D LF Control3 ==
  In3 : Inport
  In1 : Inport  Port=2
  In2 : Inport  Port=3
  In5 : Inport  Port=4
  Euler1 : Inport  Port=5
  u : Inport  Port=6
  psi1 : Inport  Port=7
  In8 : Inport  Port=8
  Add : Sum  Inputs=+-
  CA optimisation problem1 : MATLAB Function  TreatAsAtomicUnit=on
  Compensation of F_res 1 : MATLAB Function  TreatAsAtomicUnit=on
  Constant : Constant  Value=Beta_OPT
  Constant1 : Constant  Value=0
  Constant2 : Constant  Value=[CDy,Slat,S,RM,max_angle,m,g,rho_air,m_w]
  Constant3 : Constant  Value=X1
  Constant4 : Constant  Value=X1(1)  VectorParams1D=off
  Constant5 : Constant  Value=X0
  Demux1 : Demux  Outputs=3
  Demux2 : Demux  Outputs=3
  Derivative : Derivative
  Gain1 : Gain  Gain=1/cT
  Interpreted MATLAB Function2 : MATLABFcn  MATLABFcn=(30/pi*sqrt(u/4)-3000)/21000;
  MATLAB Function : MATLAB Function  TreatAsAtomicUnit=on
  MATLAB Function1 : MATLAB Function  TreatAsAtomicUnit=on
  Mux3 : Mux  Inputs=2
  Mux6 : Mux  Inputs=3
  Mux7 : Mux  Inputs=9
  Saturation1 : Saturate  UpperLimit=2*m*g  LowerLimit=0.5
  Saturation3 : Saturate  UpperLimit=max_angle  LowerLimit=-max_angle
  Saturation4 : Saturate  UpperLimit=max_angle  LowerLimit=-max_angle
  Scope{,3,5..6} (4 alike) : Scope
  Scope1 : Scope  NumInputPorts=3
  Scope2 : Scope  NumInputPorts=2
  Scope4 : Scope  NumInputPorts=2
  Sign : Signum
  Sign1 : Signum
  Terminator{1..4} (4 alike) : Terminator
  Zero-Order Hold{1..2,8..12} (7 alike) : ZeroOrderHold  SampleTime=Ts
  output1 : Outport  VectorParamsAs1DForOutWhenUnconnected=off
  Thrust_ref1 : Outport  Port=2  VectorParamsAs1DForOutWhenUnconnected=off
  output2 : Outport  Port=3  VectorParamsAs1DForOutWhenUnconnected=off
  Thrust_ref2 : Outport  Port=4  VectorParamsAs1DForOutWhenUnconnected=off
  tag scope: ExitFlag=global, Fa_zLB=global, X_mag_corr_CA=global, fval=global
  wires:
  Constant2/1 -> Mux7/4  "data"
  psi1/1 -> Mux7/7, Compensation of F_res 1/4(psi), Zero-Order Hold12/1  "psi_ref"
  Saturation1/1 -> Thrust_ref2/1, Gain1/1  "thrust_ref_N"
  Zero-Order Hold9/1 -> Mux7/6
  Mux7/1 -> CA optimisation problem1/1(data)
  [Phi_ref] -> Mux6/1  "roll_ref"
  Gain1/1 -> Interpreted MATLAB Function2/1
  Zero-Order Hold11/1 -> Mux3/1
  MATLAB Function/1(Va_G) -> Mux7/3, Scope3/1  "Va_G"
  CA optimisation problem1/1(optimized_X) -> Scope2/1, Derivative/1, output2/1, [X_mag_corr_CA]  "X_corr_CA"
  Saturation3/1 -> [Phi_ref]
  Compensation of F_res 1/2(phi_ref) -> Saturation3/1
  [Theta_ref] -> Mux6/2  "pitch_ref"
  Mux3/1 -> MATLAB Function/1(input)
  Compensation of F_res 1/1(thrust_ref) -> Saturation1/1
  Zero-Order Hold8/1 -> Mux3/2
  Euler1/1 -> Mux7/2  "F_control"
  u/1 -> Zero-Order Hold11/1  "external_wind"
  In8/1 -> Zero-Order Hold8/1  "speed_cartesian"
  In1/1 -> Zero-Order Hold10/1  "pos_sphericl"
  In5/1 -> Zero-Order Hold9/1  "quaternions"
  CA optimisation problem1/4(fval) -> [fval], Scope1/1
  CA optimisation problem1/2(F_res_spherical) -> Scope/1, [ResForces]
  CA optimisation problem1/5(exitflag) -> Scope1/2, [ExitFlag]
  CA optimisation problem1/3(Fa_zLB) -> Scope6/1, [Fa_zLB]
  [ResForces] -> Compensation of F_res 1/2(F_res_spherical)
  [Fa_zLB] -> Compensation of F_res 1/3(Fa_zLB)
  Compensation of F_res 1/3(theta_ref) -> Saturation4/1
  Saturation4/1 -> [Theta_ref]
  Constant3/1 -> MATLAB Function1/3(X1)
  Constant/1 -> MATLAB Function1/2(BETA_OPT)
  Demux1/2 -> Terminator4/1
  Zero-Order Hold2/1 -> Demux1/1
  Demux1/1 -> Terminator3/1
  Demux1/3 -> MATLAB Function1/1(betaref)  "beta_ref"
  In3/1 -> Zero-Order Hold2/1  "pos_spher_ref"
  In2/1 -> Zero-Order Hold1/1  "Euler_angles"
  Zero-Order Hold1/1 -> Demux2/1
  Demux2/2 -> Terminator2/1
  Demux2/1 -> Terminator1/1
  Mux6/1 -> output1/1  "Euler123_ref"
  Interpreted MATLAB Function2/1 -> Thrust_ref1/1  "Thrust_ref"
  Zero-Order Hold10/1 -> Compensation of F_res 1/1(pos_spherical), Mux7/1
  Zero-Order Hold12/1 -> Mux6/3  "psi_mes"
  Constant1/1 -> Compensation of F_res 1/5(psi_vicon)
  Constant5/1 -> MATLAB Function1/4(X0)
  CA optimisation problem1/6(gradient) -> Sign1/1
  Derivative/1 -> Sign/1
  Sign/1 -> Add/2, Scope4/1
  Sign1/1 -> Add/1, Scope4/2
  Add/1 -> Scope5/1
  [tether_r_ddot] -> Mux7/8
  [Twinch_PL] -> Mux7/9
  Constant4/1 -> Scope2/2, Mux7/5  "X_init"

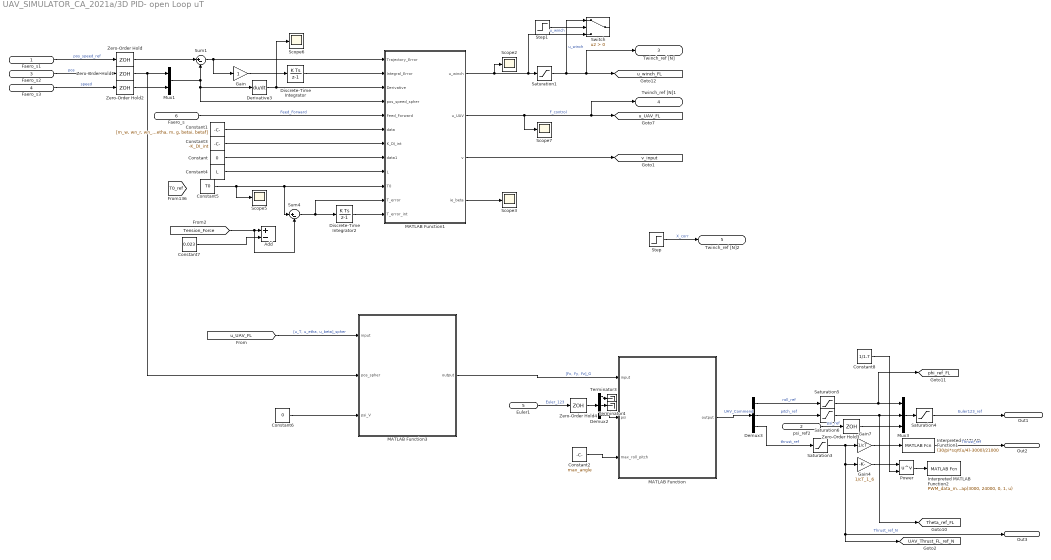
== system UAV_SIMULATOR_CA_2021a/3D PID- open Loop uT ==
  Faero_s1 : Inport
  psi_ref2 : Inport  Port=2
  Faero_s2 : Inport  Port=3
  Faero_s3 : Inport  Port=4
  Euler1 : Inport  Port=5
  Faero_s : Inport  Port=6
  Add : Sum  Inputs=+-
  Constant : Constant  Value=0
  Constant1 : Constant  Value=[m_w, wn_r, wn_beta, wn_etha, m, g, betai, betaf]
  Constant2 : Constant  Value=max_angle
  Constant3 : Constant  Value=-K_DI_int
  Constant4 : Constant  Value=L
  Constant5 : Constant  Value=T0
  Constant6 : Constant  Value=0
  Constant7 : Constant  Value=0.023
  Constant8 : Constant  Value=1/1.7
  Demux2 : Demux  Outputs=3
  Demux3 : Demux  Outputs=3
  Derivative3 : Derivative
  Discrete-Time Integrator : DiscreteIntegrator  SampleTime=Ts  ICPrevOutput=DiscIntNeverNeededParam  ICPrevScaledInput=DiscIntNeverNeededParam
  Discrete-Time Integrator2 : DiscreteIntegrator  SampleTime=Ts  ICPrevOutput=DiscIntNeverNeededParam  ICPrevScaledInput=DiscIntNeverNeededParam
  Gain : Gain
  Gain4 : Gain  Gain=1/cT_1_6
  Gain7 : Gain  Gain=1/cT
  Interpreted MATLAB Function1 : MATLABFcn  MATLABFcn=(30/pi*sqrt(u/4)-3000)/21000
  Interpreted MATLAB Function2 : MATLABFcn  MATLABFcn=PWM_data_map(3000, 24000, 0, 1, u)
  MATLAB Function : MATLAB Function  TreatAsAtomicUnit=on
  MATLAB Function1 : MATLAB Function  TreatAsAtomicUnit=on
  MATLAB Function3 : MATLAB Function  TreatAsAtomicUnit=on
  Mux1 : Mux  Inputs=2
  Mux3 : Mux  Inputs=3
  Power : Math  Operator=pow
  Saturation1 : Saturate  UpperLimit=6.2  LowerLimit=0.06
  Saturation3 : Saturate  UpperLimit=2*m*g  LowerLimit=0
  Saturation4 : Saturate  UpperLimit=[max_angle max_angle 200*pi]  LowerLimit=-[max_angle max_angle 200*pi]
  Saturation5 : Saturate  UpperLimit=max_angle  LowerLimit=-max_angle
  Saturation6 : Saturate  UpperLimit=max_angle  LowerLimit=-max_angle
  Scope{2..3,5..7} (5 alike) : Scope
  Step : Step  Time=0  After=4.3  SampleTime=0
  Step1 : Step  Time=30  Before=1  After=0  SampleTime=0
  Sum1 : Sum  Inputs=|+-
  Sum4 : Sum  Inputs=|+-
  Switch : Switch  Criteria=u2 > Threshold  SaturateOnIntegerOverflow=off  InputSameDT=off
  Terminator3 : Terminator
  Terminator4 : Terminator
  Zero-Order Hold{,1..4} (5 alike) : ZeroOrderHold  SampleTime=Ts
  Out1 : Outport  VectorParamsAs1DForOutWhenUnconnected=off
  Out2 : Outport  Port=2  VectorParamsAs1DForOutWhenUnconnected=off
  Twinch_ref [N] : Outport  Port=3
  Twinch_ref [N]1 : Outport  Port=4
  Twinch_ref [N]2 : Outport  Port=5
  Out3 : Outport  Port=6  VectorParamsAs1DForOutWhenUnconnected=off
  tag scope: Theta_ref_FL=global, UAV_Thrust_FL_ref_N=global, phi_ref_FL=global, u_UAV_FL=global, u_winch_FL=global, v_input=global
  wires:
  Step/1 -> Twinch_ref [N]2/1  "X_corr"
  Faero_s3/1 -> Zero-Order Hold2/1  "speed"
  Discrete-Time Integrator/1 -> MATLAB Function1/2(Integral_Error)
  Faero_s1/1 -> Zero-Order Hold/1  "pos_speed_ref"
  Faero_s2/1 -> Zero-Order Hold1/1  "pos"
  Derivative3/1 -> Scope6/1, MATLAB Function1/3(Derivative)
  Mux1/1 -> Derivative3/1, MATLAB Function1/4(pos_speed_spher), Sum1/2
  Faero_s/1 -> MATLAB Function1/5(Feed_Forward)  "Feed_Forward"
  Constant1/1 -> MATLAB Function1/6(data)
  MATLAB Function1/2(u_UAV) -> Scope7/1, Twinch_ref [N]1/1, [u_UAV_FL]  "F_control"
  Euler1/1 -> Zero-Order Hold4/1  "Euler_123"
  Demux2/1 -> Terminator3/1
  Demux2/2 -> Terminator4/1
  Constant2/1 -> MATLAB Function/3(max_roll_pitch)
  Saturation3/1 -> Gain7/1, Gain4/1, Out3/1, [UAV_Thrust_FL_ref_N]  "Thrust_ref_N"
  Saturation6/1 -> [Theta_ref_FL], Mux3/2
  Demux3/3 -> Saturation3/1  "thrust_ref"
  Demux3/1 -> Saturation5/1  "roll_ref"
  psi_ref2/1 -> Zero-Order Hold3/1  "psi_ref"
  Mux3/1 -> Saturation4/1
  Demux3/2 -> Saturation6/1  "pitch_ref"
  Saturation5/1 -> Mux3/1, [phi_ref_FL]
  Gain7/1 -> Interpreted MATLAB Function1/1
  Interpreted MATLAB Function1/1 -> Out2/1  "Thrust_ref"
  Saturation4/1 -> Out1/1  "Euler123_ref"
  MATLAB Function/1(output) -> Demux3/1  "UAV_Commend"
  MATLAB Function1/3(v) -> [v_input]
  MATLAB Function1/4(ie_beta) -> Scope3/1
  Sum1/1 -> Gain/1, MATLAB Function1/1(Trajectory_Error)
  Constant3/1 -> MATLAB Function1/7(K_DI_int)
  Constant4/1 -> MATLAB Function1/9(L)
  Zero-Order Hold/1 -> Sum1/1
  Zero-Order Hold1/1 -> MATLAB Function3/2(pos_spher), Mux1/1
  Zero-Order Hold2/1 -> Mux1/2
  Zero-Order Hold4/1 -> Demux2/1
  MATLAB Function3/1(output) -> MATLAB Function/1(input)  "[Fx, Fy, Fz]_G"
  Constant/1 -> MATLAB Function1/8(data1)
  Gain/1 -> Discrete-Time Integrator/1
  [u_UAV_FL] -> MATLAB Function3/1(input)  "[u_T, u_etha, u_beta]_spher"
  Zero-Order Hold3/1 -> Mux3/3
  Constant6/1 -> MATLAB Function3/3(psi_V)
  Demux2/3 -> MATLAB Function/2(psi)
  Constant5/1 -> Scope5/1, Sum4/1, MATLAB Function1/10(T0)
  Sum4/1 -> MATLAB Function1/11(T_error), Discrete-Time Integrator2/1
  Discrete-Time Integrator2/1 -> MATLAB Function1/12(T_error_int)
  Constant7/1 -> Add/2
  [Tension_Force] -> Sum4/2, Add/1
  Gain4/1 -> Power/1
  Constant8/1 -> Power/2
  Power/1 -> Interpreted MATLAB Function2/1
  MATLAB Function1/1(u_winch) -> Saturation1/1, Switch/3, Scope2/1  "u_winch"
  Step1/1 -> Switch/2
  Saturation1/1 -> Twinch_ref [N]/1, [u_winch_FL], Switch/1  "u_winch"

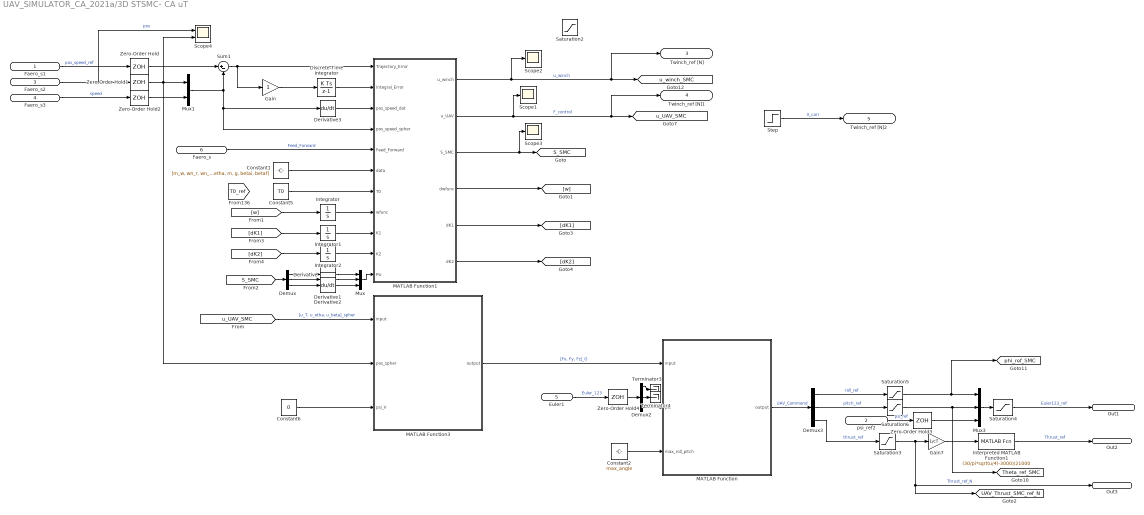
== system UAV_SIMULATOR_CA_2021a/3D STSMC- CA uT ==
  Faero_s1 : Inport
  psi_ref2 : Inport  Port=2
  Faero_s2 : Inport  Port=3
  Faero_s3 : Inport  Port=4
  Euler1 : Inport  Port=5
  Faero_s : Inport  Port=6
  Constant1 : Constant  Value=[m_w, wn_r, wn_beta, wn_etha, m, g, betai, betaf]
  Constant2 : Constant  Value=max_angle
  Constant5 : Constant  Value=T0
  Constant6 : Constant  Value=0
  Demux : Demux  Outputs=3
  Demux2 : Demux  Outputs=3
  Demux3 : Demux  Outputs=3
  Derivative{,1..3} (4 alike) : Derivative
  Discrete-Time Integrator : DiscreteIntegrator  SampleTime=Ts  ICPrevOutput=DiscIntNeverNeededParam  ICPrevScaledInput=DiscIntNeverNeededParam
  Gain : Gain
  Gain7 : Gain  Gain=1/cT
  Integrator : Integrator  InitialCondition=[0;0;0]
  Integrator1 : Integrator  InitialCondition=[0;0;0]
  Integrator2 : Integrator  InitialCondition=[0;0;0]
  Interpreted MATLAB Function1 : MATLABFcn  MATLABFcn=(30/pi*sqrt(u/4)-3000)/21000
  MATLAB Function : MATLAB Function  TreatAsAtomicUnit=on
  MATLAB Function1 : MATLAB Function  TreatAsAtomicUnit=on
  MATLAB Function3 : MATLAB Function  TreatAsAtomicUnit=on
  Mux : Mux  Inputs=3
  Mux1 : Mux  Inputs=2
  Mux3 : Mux  Inputs=3
  Saturation2 : Saturate  UpperLimit=6  LowerLimit=0.06
  Saturation3 : Saturate  UpperLimit=2*m*g  LowerLimit=0
  Saturation4 : Saturate  UpperLimit=[max_angle max_angle 200*pi]  LowerLimit=-[max_angle max_angle 200*pi]
  Saturation5 : Saturate  UpperLimit=max_angle  LowerLimit=-max_angle
  Saturation6 : Saturate  UpperLimit=max_angle  LowerLimit=-max_angle
  Scope1 : Scope
  Scope2 : Scope
  Scope3 : Scope
  Scope4 : Scope  NumInputPorts=2
  Step : Step  Time=0  After=4  SampleTime=0
  Sum1 : Sum  Inputs=|+-
  Terminator3 : Terminator
  Terminator4 : Terminator
  Zero-Order Hold{,1..4} (5 alike) : ZeroOrderHold  SampleTime=Ts
  Out1 : Outport  VectorParamsAs1DForOutWhenUnconnected=off
  Out2 : Outport  Port=2  VectorParamsAs1DForOutWhenUnconnected=off
  Twinch_ref [N] : Outport  Port=3
  Twinch_ref [N]1 : Outport  Port=4
  Twinch_ref [N]2 : Outport  Port=5
  Out3 : Outport  Port=6  VectorParamsAs1DForOutWhenUnconnected=off
  tag scope: S_SMC=global, Theta_ref_SMC=global, UAV_Thrust_SMC_ref_N=global, phi_ref_SMC=global, u_UAV_SMC=global, u_winch_SMC=global
  wires:
  Step/1 -> Twinch_ref [N]2/1  "X_corr"
  Faero_s3/1 -> Zero-Order Hold2/1  "speed"
  Discrete-Time Integrator/1 -> MATLAB Function1/2(Integral_Error)
  Faero_s1/1 -> Zero-Order Hold/1  "pos_speed_ref"
  Faero_s2/1 -> Scope4/1, Zero-Order Hold1/1  "pos"
  Derivative3/1 -> MATLAB Function1/3(pos_speed_dot)
  Mux1/1 -> Derivative3/1, MATLAB Function1/4(pos_speed_spher), Sum1/2
  Faero_s/1 -> MATLAB Function1/5(Feed_Forward)  "Feed_Forward"
  Constant1/1 -> MATLAB Function1/6(data)
  MATLAB Function1/2(u_UAV) -> Scope1/1, Twinch_ref [N]1/1, [u_UAV_SMC]  "F_control"
  Euler1/1 -> Zero-Order Hold4/1  "Euler_123"
  Demux2/1 -> Terminator3/1
  Demux2/2 -> Terminator4/1
  Constant2/1 -> MATLAB Function/3(max_roll_pitch)
  Saturation3/1 -> Gain7/1, Out3/1, [UAV_Thrust_SMC_ref_N]  "Thrust_ref_N"
  Saturation6/1 -> [Theta_ref_SMC], Mux3/2
  Demux3/3 -> Saturation3/1  "thrust_ref"
  Demux3/1 -> Saturation5/1  "roll_ref"
  psi_ref2/1 -> Zero-Order Hold3/1  "psi_ref"
  Mux3/1 -> Saturation4/1
  Demux3/2 -> Saturation6/1  "pitch_ref"
  Saturation5/1 -> Mux3/1, [phi_ref_SMC]
  Gain7/1 -> Interpreted MATLAB Function1/1
  Interpreted MATLAB Function1/1 -> Out2/1  "Thrust_ref"
  Saturation4/1 -> Out1/1  "Euler123_ref"
  MATLAB Function/1(output) -> Demux3/1  "UAV_Commend"
  MATLAB Function1/3(S_SMC) -> Scope3/1, [S_SMC]
  Sum1/1 -> Gain/1, MATLAB Function1/1(Trajectory_Error)
  Zero-Order Hold/1 -> Sum1/1
  Zero-Order Hold1/1 -> MATLAB Function3/2(pos_spher), Scope4/2, Mux1/1
  Zero-Order Hold2/1 -> Mux1/2
  Zero-Order Hold4/1 -> Demux2/1
  MATLAB Function3/1(output) -> MATLAB Function/1(input)  "[Fx, Fy, Fz]_G"
  MATLAB Function1/1(u_winch) -> Twinch_ref [N]/1, [u_winch_SMC], Scope2/1  "u_winch"
  Gain/1 -> Discrete-Time Integrator/1
  [u_UAV_SMC] -> MATLAB Function3/1(input)  "[u_T, u_etha, u_beta]_spher"
  Zero-Order Hold3/1 -> Mux3/3
  Constant6/1 -> MATLAB Function3/3(psi_V)
  Demux2/3 -> MATLAB Function/2(psi)
  Constant5/1 -> MATLAB Function1/7(T0)
  MATLAB Function1/4(dwfunc) -> [w]
  [w] -> Integrator/1
  Integrator/1 -> MATLAB Function1/8(wfunc)
  Demux/1 -> Derivative/1
  Mux/1 -> MATLAB Function1/11(Psi)
  MATLAB Function1/5(dK1) -> [dK1]
  Integrator1/1 -> MATLAB Function1/9(K1)
  [dK1] -> Integrator1/1
  [dK2] -> Integrator2/1
  Integrator2/1 -> MATLAB Function1/10(K2)
  MATLAB Function1/6(dK2) -> [dK2]
  [S_SMC] -> Demux/1
  Demux/2 -> Derivative1/1
  Demux/3 -> Derivative2/1
  Derivative/1 -> Mux/1
  Derivative1/1 -> Mux/2
  Derivative2/1 -> Mux/3

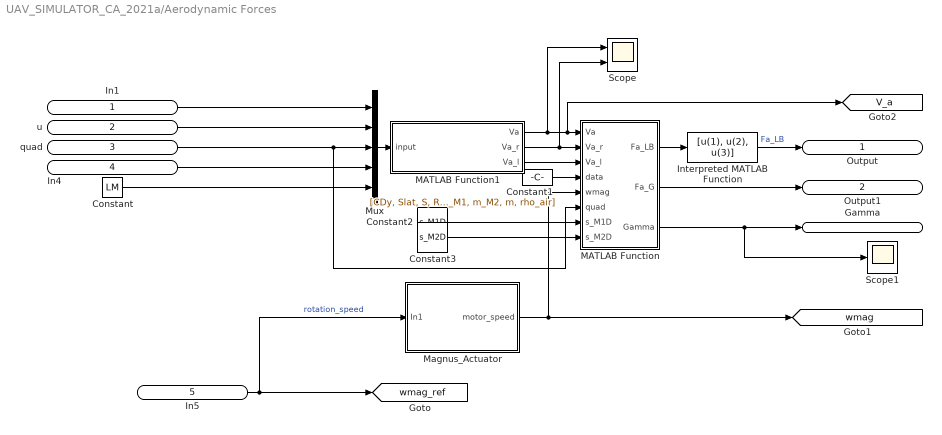
== system UAV_SIMULATOR_CA_2021a/Aerodynamic Forces ==
  In1 : Inport
  u : Inport  Port=2
  quad : Inport  Port=3
  In4 : Inport  Port=4
  In5 : Inport  Port=5
  Constant : Constant  Value=LM
  Constant1 : Constant  Value=[CDy, Slat, S, RM, LM, m_M1, m_M2, m, rho_air]
  Constant2 : Constant  Value=s_M1D
  Constant3 : Constant  Value=s_M2D
  Interpreted MATLAB Function : MATLABFcn  MATLABFcn=[u(1), u(2), u(3)]
  MATLAB Function : MATLAB Function  TreatAsAtomicUnit=on
  MATLAB Function1 : MATLAB Function  TreatAsAtomicUnit=on
  Magnus_Actuator : Subsystem
  Mux : Mux  Inputs=5
  Scope : Scope  NumInputPorts=2
  Scope1 : Scope
  Output : Outport
  Output1 : Outport  Port=2
  Gamma : Outport  Port=3
  tag scope: V_a=global, wmag=global, wmag_ref=global
  wires:
  Magnus_Actuator/1(motor_speed) -> MATLAB Function/5(wmag), [wmag]
  MATLAB Function/2(Fa_G) -> Output1/1
  quad/1 -> MATLAB Function/6(quad), Mux/3
  u/1 -> Mux/2
  MATLAB Function/1(Fa_LB) -> Interpreted MATLAB Function/1
  Interpreted MATLAB Function/1 -> Output/1  "Fa_LB"
  MATLAB Function1/1(Va) -> Scope/1, [V_a], MATLAB Function/1(Va)
  Constant1/1 -> MATLAB Function/4(data)
  Mux/1 -> MATLAB Function1/1(input)
  In4/1 -> Mux/4
  In1/1 -> Mux/1
  Constant/1 -> Mux/5
  MATLAB Function1/2(Va_r) -> Scope/2, MATLAB Function/2(Va_r)
  MATLAB Function1/3(Va_l) -> MATLAB Function/3(Va_l)
  MATLAB Function/3(Gamma) -> Scope1/1, Gamma/1
  Constant2/1 -> MATLAB Function/7(s_M1D)
  Constant3/1 -> MATLAB Function/8(s_M2D)
  In5/1 -> [wmag_ref], Magnus_Actuator/1(In1)  "rotation_speed"

== system UAV_SIMULATOR_CA_2021a/ROUTEUR1 ==
  In1 : Inport
  In2 : Inport  Port=2
  Delay2 : Delay  DelayLength=3  SampleTime=Ts
  Demux : Demux
  Manual Switch : ManualSwitch  CurrentSetting=0
  Mux : Mux  Inputs=2
  Mux1 : Mux  Inputs=3
  PQR_ref : Outport  VectorParamsAs1DForOutWhenUnconnected=off
  PQR_ref1 : Outport  Port=2  VectorParamsAs1DForOutWhenUnconnected=off
  wires:
  In1/1 -> Mux/1  "Euler123_ref"
  In2/1 -> Mux/2  "Thrust_ref"
  Mux/1 -> Delay2/1, Manual Switch/1
  Demux/4 -> PQR_ref1/1  "Thrust_ref_wifi"
  Demux/1 -> Mux1/1
  Demux/2 -> Mux1/2
  Demux/3 -> Mux1/3
  Mux1/1 -> PQR_ref/1  "Euler123_ref_wifi"
  Delay2/1 -> Manual Switch/2
  Manual Switch/1 -> Demux/1

== system UAV_SIMULATOR_CA_2021a/Subsystem1 ==
  Derivative4 : Derivative
  Mux6 : Mux  Inputs=2
  Mux8 : Mux  Inputs=3
  beta_ref : Subsystem
  etha_ref1 : Subsystem
  r_ref : Subsystem
  spherical_ref : Outport
  wires:
  Derivative4/1 -> Mux6/2  "dw"
  Mux8/1 -> Derivative4/1, Mux6/1  "w"
  Mux6/1 -> spherical_ref/1
  beta_ref/1(beta-ref) -> Mux8/3
  etha_ref1/1(beta-ref) -> Mux8/2
  r_ref/1(r_ref) -> Mux8/1

== system UAV_SIMULATOR_CA_2021a/Subsystem2 ==
  y : Inport
  control : Inport  Port=2
  Thrust_ref : Inport  Port=3
  euler_ref : Inport  Port=4
  cov : Inport  Port=5
  Add1 : Sum
  Constant1 : Constant  Value=[m_w, m, g]
  Constant2 : Constant  Value=[m_w, m, g, Ts]
  Constant3 : Constant
  MATLAB Function1 : MATLAB Function  TreatAsAtomicUnit=on
  MATLAB Function2 : MATLAB Function  TreatAsAtomicUnit=on
  Noice on Covariance : MATLAB Function  TreatAsAtomicUnit=on
  Unit Delay : UnitDelay  InitialCondition=eye(9)  SampleTime=Ts  HasFrameUpgradeWarning=on
  Unit Delay1 : UnitDelay  InitialCondition=[ri;0;ethai;0;betai;0;Fa_L_int]  SampleTime=Ts  HasFrameUpgradeWarning=on
  x_est : Outport
  Cov : Outport  Port=2
  wires:
  MATLAB Function1/2(Cov1) -> Unit Delay/1
  Noice on Covariance/1(y) -> Add1/2
  Constant3/1 -> Noice on Covariance/1(u)
  Constant1/1 -> MATLAB Function2/3(data)
  Constant2/1 -> MATLAB Function1/7(data)
  cov/1 -> MATLAB Function1/4(Cov)  "covarianc"
  MATLAB Function1/1(x_est) -> Unit Delay1/1
  Unit Delay/1 -> Cov/1  "covariance"
  Unit Delay1/1 -> x_est/1, MATLAB Function1/2(pos_updated), MATLAB Function2/1(x_e)  "position_estimated"
  control/1 -> MATLAB Function2/2(control)  "control_signals"
  euler_ref/1 -> MATLAB Function1/6(euler_angles)  "Euler_angles"
  Thrust_ref/1 -> MATLAB Function1/5(Thrust)  "Thrust_Force_N"
  MATLAB Function2/1(xdot_e) -> MATLAB Function1/3(speed), Add1/1
  y/1 -> MATLAB Function1/1(y)  "measurments"
